simulink model "mho_distance_model"  (R2025a)
settings: Solver=FixedStepDiscrete  StartTime=0.0  StopTime=1.2  FixedStep=5e-05  RelTol=1e-3
libraries: spsThreePhasePISectionLineLib x2, spsThreePhaseBreakerLib x1, spsThreePhaseFaultLib x1, spsThreePhaseSeriesRLCLoadLib x1, spsThreePhaseSourceLib x1, spsThreePhaseVIMeasurementLib x1, sps_lib x1
settings Model: Creator=panka  LastModifiedBy=panka

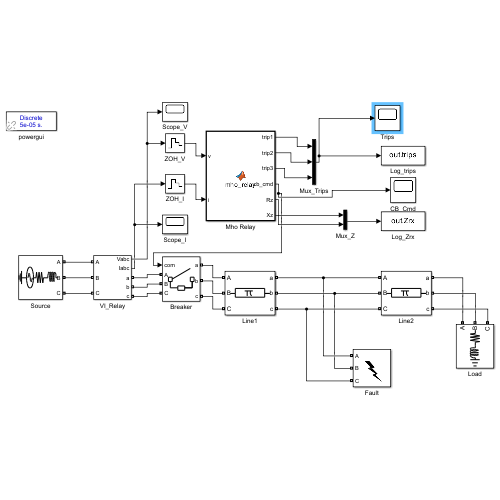
[thumbnail: Simulink's stored preview of the top-level diagram]
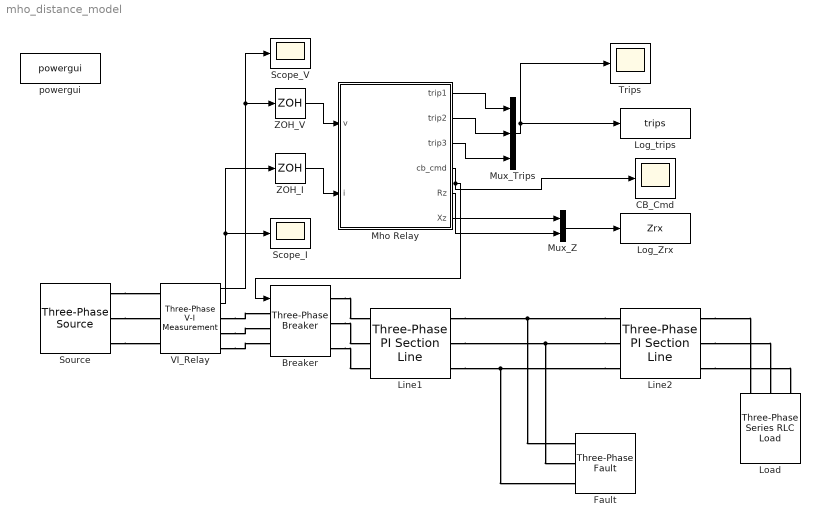
== system mho_distance_model ==
  Breaker : spsThreePhaseBreakerLib/Three-Phase Breaker  InitialState=open  SwitchA=on  SwitchB=on  SwitchC=on  SwitchTimes="[1/60  5/60]"  External=on  BreakerResistance=0.001  SnubberResistance=1e6  SnubberCapacitance=inf  Measurements=None
  CB_Cmd : Scope
      settings: ActiveDisplayYMinimum=-0.12499999999999997  ActiveDisplayYMaximum=1.125
  Fault : spsThreePhaseFaultLib/Three-Phase Fault  InitialStates=0  FaultA=on  FaultB=off  FaultC=off  GroundFault=on  SwitchTimes=[0.4 2.2]  External=off  SwitchStatus=NaN  FaultResistance=0.01  GroundResistance=0.01  SnubberResistance=1e6  SnubberCapacitance=inf  Measurements=None
  Line1 : spsThreePhasePISectionLineLib/Three-Phase PI Section Line  LConnTagsString=a|b|c  RConnTagsString=A|B|C  Length=60  Frequency=50  Resistances=[0.01273 0.3864]  Inductances=[0.0009337 0.0041264]  Capacitances=[1.274e-08 7.751e-09]
  Line2 : spsThreePhasePISectionLineLib/Three-Phase PI Section Line  LConnTagsString=a|b|c  RConnTagsString=A|B|C  Length=90  Frequency=50  Resistances=[0.01273 0.3864]  Inductances=[0.0009337 0.0041264]  Capacitances=[1.274e-08 7.751e-09]
  Load : spsThreePhaseSeriesRLCLoadLib/Three-Phase Series RLC Load  LConnTagsString=A|B|C  Configuration=Y (grounded)  NominalVoltage=220000  Vabc=[1e3 1e3 1e3]  Vabcp=[1e3 1e3 1e3]  NominalFrequency=50  UnbalancedPower=off  ActivePower=100e6  InductivePower=20e6  CapacitivePower=0  Pabc=[10e3 9e3 11e3]  QLabc=[100 90 110]  QCabc=[100 90 110]  Pabcp=[10e3 9e3 11e3]  QLabcp=[100 90 110]  QCabcp=[100 90 110]  Measurements=None  LoadType=constant Z
  Log_Zrx : ToWorkspace  VariableName=Zrx  SaveFormat=Timeseries  SampleTime=-1
  Log_trips : ToWorkspace  VariableName=trips  SaveFormat=Timeseries  SampleTime=-1
  Mho Relay : MATLAB Function  TreatAsAtomicUnit=on
  Mux_Trips : Mux  Inputs=3
  Mux_Z : Mux  Inputs=2
  Scope_I : Scope
      settings: ActiveDisplayYMinimum=-1697.5055862923259  ActiveDisplayYMaximum=6904.7302111290965
  Scope_V : Scope
      settings: ActiveDisplayYMinimum=-353825.82712748589  ActiveDisplayYMaximum=319445.62225979165
  Source : spsThreePhaseSourceLib/Three-Phase Source  InternalConnection=Yg  VoltagePhases=off  Voltage=220000  PhaseAngle=0  Voltage_phases=[25e3 25e3 25e3]/sqrt(3)  PhaseAngles_phases=[0 -120 +120]  Frequency=50  NonIdealSource=on  SpecifyImpedance=on  Resistance=0.8929  Inductance=16.58e-3  ShortCircuitLevel=5e9  BaseVoltage=220000  XRratio=10  BusType=swing  Pref=10e3  Qref=0  Prefabc=[10e3, 10e3, 10e3]  Qrefabc=[0, 0, 0]  Qmin=-inf  Qmax=inf
  Trips : Scope
      settings: ActiveDisplayYMinimum=-0.12499999999999997  ActiveDisplayYMaximum=1.125
  VI_Relay : spsThreePhaseVIMeasurementLib/Three-Phase V-I Measurement  VoltageMeasurement=phase-to-ground  SetLabelV=off  LabelV=Vabc  Vpu=off  VpuLL=off  CurrentMeasurement=yes  SetLabelI=off  LabelI=Iabc  Ipu=off  Pbase=100e6  Vbase=500e3  OutputType=Complex  PhasorSimulation=off  PSBequivalent=0
  ZOH_I : ZeroOrderHold  SampleTime=0.0002
  ZOH_V : ZeroOrderHold  SampleTime=0.0002
  powergui : sps_lib/powergui  Priority=1  SimulationMode=Discrete  SampleTime=5e-05  frequency=60  Iterations=50  frequencyindice=50  Pbase=100e6  ErrMax=1e-4  UnitsV=kV  UnitsW=MW  buscounter=0  FunctionMessages=off  echomessages=off  EnableUseOfTLC=off  CurrentSourceSwitches=off  DisableSnubberDevices=off  DisableRonSwitches=off  DisableVfSwitches=off  DisplayEquations=off  AutomaticDiscreteSolvers=off  SolverType=Tustin/Backward Euler (TBE)  Interpol=off  ExternalGateDelay=off  methode=off  Ts=100  x0status=blocks  SPID=on  SwTol=0  HookPort=off  NonlinearTolerance=1e-4  nMaxIteration=100  ContinueOnMaxIteration=off  RestoreLinks=warning  ResistiveCurrentMeasurement=off  Frange=[0:2:500]  Ylog=off  Xlog=on  ShowGrid=off  save=off  variable=ZData  structure=0  ZoomFFT=off  StartTime=0.0  cycles=1  DisplayStyle=1  fundamental=60  FreqAxis=off  MaxFrequency=1000  frequencyindicesteady=1  RmsSteady=1  display=off
  wires:
  VI_Relay/1 -> ZOH_V/1, Scope_V/1
  VI_Relay/2 -> ZOH_I/1, Scope_I/1
  ZOH_V/1 -> Mho Relay/1(v)
  ZOH_I/1 -> Mho Relay/2(i)
  Mho Relay/1(trip1) -> Mux_Trips/1
  Mho Relay/2(trip2) -> Mux_Trips/2
  Mho Relay/3(trip3) -> Mux_Trips/3
  Mux_Trips/1 -> Trips/1, Log_trips/1
  Mho Relay/4(cb_cmd) -> CB_Cmd/1, Breaker/1
  Mho Relay/5(Rz) -> Mux_Z/1
  Mho Relay/6(Xz) -> Mux_Z/2
  Mux_Z/1 -> Log_Zrx/1
  connections:
  Source/RConn1 -- VI_Relay/LConn1
  Source/RConn2 -- VI_Relay/LConn2
  Source/RConn3 -- VI_Relay/LConn3
  VI_Relay/RConn1 -- Breaker/LConn1
  VI_Relay/RConn2 -- Breaker/LConn2
  VI_Relay/RConn3 -- Breaker/LConn3
  Breaker/RConn1 -- Line1/LConn1
  Breaker/RConn2 -- Line1/LConn2
  Breaker/RConn3 -- Line1/LConn3
  Line2/LConn1 -- Fault/LConn1 -- Line1/RConn1
  Line2/LConn2 -- Line1/RConn2 -- Fault/LConn2
  Line2/LConn3 -- Line1/RConn3 -- Fault/LConn3
  Line2/RConn1 -- Load/LConn1
  Line2/RConn2 -- Load/LConn2
  Line2/RConn3 -- Load/LConn3

== matlab function mho_distance_model/Mho Relay ==
  data: v input; trip1 output; i input; trip2 output; trip3 output; cb_cmd output; Rz output; Xz output
function [trip1,trip2,trip3,cb_cmd,Rz,Xz] = mho_relay(v,i)
%#codegen
N = 100; Ts = 0.0002;
kN = complex(1.15605303,-0.374458535);
th = 1.5274254;
Zr = [23.4885284 35.2327926 44.0409908];
Tz = [0 0.3 0.6];
persistent bv bi n t2 t3 l1 l2 l3
if isempty(bv)
    bv = zeros(N,3); bi = zeros(N,3); n = 0; t2 = 0; t3 = 0;
    l1 = false; l2 = false; l3 = false;
end
trip1 = double(l1); trip2 = double(l2); trip3 = double(l3);
cb_cmd = double(~(l1 || l2 || l3));
Rz = NaN; Xz = NaN;
bv = [bv(2:end,:); reshape(v,1,3)];
bi = [bi(2:end,:); reshape(i,1,3)];
n = min(n + 1, N);
if n < N
    return;
end
w  = exp(-1j*2*pi*(0:N-1)'/N);
V  = (sqrt(2)/N)*(bv.'*w);
I  = (sqrt(2)/N)*(bi.'*w);
Ir = I(1)+I(2)+I(3);
Vl = [V(1); V(2); V(3); V(1)-V(2); V(2)-V(3); V(3)-V(1)];
Il = [I(1)+kN*Ir; I(2)+kN*Ir; I(3)+kN*Ir; I(1)-I(2); I(2)-I(3); I(3)-I(1)];
Z  = complex(1e6*ones(6,1),0);
for k = 1:6
    if abs(Il(k)) > 50
        Z(k) = Vl(k)/Il(k);
    end
end
[zm,idx] = min(abs(Z));
if zm < 1e5
    Rz = real(Z(idx)); Xz = imag(Z(idx));
end
in1 = false; in2 = false; in3 = false;
for k = 1:6
    in1 = in1 || (abs(Z(k) - 0.5*Zr(1)*exp(1j*th)) < 0.5*Zr(1));
    in2 = in2 || (abs(Z(k) - 0.5*Zr(2)*exp(1j*th)) < 0.5*Zr(2));
    in3 = in3 || (abs(Z(k) - 0.5*Zr(3)*exp(1j*th)) < 0.5*Zr(3));
end
if in2, t2 = t2 + Ts; else, t2 = 0; end
if in3, t3 = t3 + Ts; else, t3 = 0; end
if in1 && Tz(1) <= 0, l1 = true; end
if in2 && t2 >= Tz(2), l2 = true; end
if in3 && t3 >= Tz(3), l3 = true; end
trip1 = double(l1); trip2 = double(l2); trip3 = double(l3);
cb_cmd = double(~(l1 || l2 || l3));
end
